simulink model "gtm_design_lpv"  (R2021b)
settings: Solver=VariableStepAuto  StartTime=0.0  StopTime=10  FixedStep=0.005  MaxStep=0.005  RelTol=1e-3
StopFcn:
  | MWSout=grabmws(bdroot);
  | MWSout.lastrun=datestr(now);
values from neighbouring files (symbols this model uses):
  s = tf('s')    [SingleDOF.m]    (also in main.m; mainSimple.m; newmain.m)
undefined symbols (not defined in the file or in its folder): Aero, aftfuel, aftfuel_pos, AILL, AILLC, AILR, AILRC, alpha_deg, altitude_ft, Ax_g, Ay_g, Az_g, b, beta_deg, bias, BRAKEC, Cbar, cg_pos0, cg_shift_gear, DamageCase, DamageModels, DamageOnsetTime, Earth, ELLIB, ELLIBC, ELLOB, ELLOBC, ELRIB, ELRIBC, ELROB, ELROBC, engl_ang, engl_pos, engr_ang, engr_pos, FLAPLIB, FLAPLIC, FLAPLOB, FLAPLOC, FLAPRIB, FLAPRIC, FLAPROB, FLAPROC, ft, FuelUsed_Init, fwdfuel, fwdfuel_pos, GEAR, GEARC, Inertia0, Inertia_shift_gear, Ixx_model, Iyy_model, Izz_model, KTAS, LandingGear, LengON, LinearizeModeOn, NAV_altitude_m, NAV_latitude_deg ... (+51)
libraries: simulink_extras x63, simulink_need_slupdate x30, LPVBlockLibrary x20, aerolibconvert2 x6, aerolibtransform2 x5, uavalgslib x4, UserContent_lib x3, simulink x3, robotcorelib x1, uavutilslib x1
(part 3 of 8)

== system gtm_design_lpv/Subsystem2/LPV1 ==
  Guidance : Inport
  Feedback : Inport  Port=2
  Add : Sum
  Bus Selector : BusSelector  OutputSignals=AirData.KTAS,AirData.altitude_ft,SurfacePos.AILL,SurfacePos.AILR
  Bus Selector3 : BusSelector  OutputSignals=An_c  OutputAsBus=on
  Bus Selector4 : BusSelector  OutputSignals=beta_c,phi_c  OutputAsBus=on
  Bus Selector5 : BusSelector  OutputSignals=AirData.alpha_deg,MAG3.q_deg,MAG3.Az_g
  Bus Selector6 : BusSelector  OutputSignals=AirData.beta_deg,MAG3.p_deg,MAG3.r_deg,MIDG.phi_deg,MAG3.Ay_g
  Bus to Vector : BusToVector
  Bus to Vector1 : BusToVector
  Constant : Constant
  Degrees to Radians{,1..5} (6 alike) : simulink_extras/Transformations/Degrees to Radians
  Demux1 : Demux  Outputs=2
  Gain : Gain  Gain=1/2
  Gain1 : Gain  Gain=1/100
  Gain2 : Gain  Gain=32.17405
  Gain3 : Gain  Gain=32.17405
  Gain4 : Gain  Gain=100
  Gain5 : Gain  Gain=100
  LPVBlock1 : LPVBlockLibrary/LPVBlock  sys=K_lon_lpv  plist={'rho1_tas_param';'rho2_alt_param';'rho3_mor_param'}  x0=0
      settings: SourceProductName=LPVTools Blocks
  LPVBlock2 : LPVBlockLibrary/LPVBlock  sys=K_lat_lpv  plist={'rho1_tas_param';'rho2_alt_param';'rho3_mor_param'}  x0=0
      settings: SourceProductName=LPVTools Blocks
  LPVBlock3 : LPVBlockLibrary/LPVBlock  sys=sch_alp_trim  plist={'rho1_tas_param';'rho2_alt_param';'rho3_mor_param'}  x0=0
      settings: SourceProductName=LPVTools Blocks
  Mux : Mux  Inputs=3
  Mux4 : Mux  Inputs=3
  Mux5 : Mux  Inputs=2
  Mux6 : Mux  Inputs=5
  Mux7 : Mux  Inputs=2
  Mux8 : Mux
  Radians to Degrees : simulink_extras/Transformations/Radians to Degrees
  Radians to Degrees1 : simulink_extras/Transformations/Radians to Degrees
  Selector : Selector  InputPortWidth=3  IndexOptions=Index vector (dialog)  Indices=3  OutputSizes=1
  Sum : Sum  Inputs=|+-
  Sum1 : Sum  Inputs=++|
  Sum2 : Sum  Inputs=|+-
  Out : Outport  InitialOutput=zeros(4,1)
  wires:
  Mux8/1 -> Out/1
  Radians to Degrees1/1 -> Mux8/1
  Gain4/1 -> Mux8/2
  Gain5/1 -> Mux8/3
  Radians to Degrees/1 -> Mux8/4
  Demux1/2 -> Radians to Degrees/1
  Sum1/1 -> Gain5/1
  Sum2/1 -> Gain4/1
  Demux1/1 -> Sum2/1, Sum1/2
  Selector/1 -> Sum2/2, Sum1/1
  [rho] -> Selector/1
  LPVBlock1/1 -> Radians to Degrees1/1
  LPVBlock2/1 -> Demux1/1
  [rho] -> LPVBlock2/2
  Mux7/1 -> LPVBlock2/1
  Bus to Vector1/1 -> Mux7/1
  Mux6/1 -> Mux7/2
  Degrees to Radians5/1 -> Mux6/4
  Degrees to Radians4/1 -> Mux6/3
  Degrees to Radians3/1 -> Mux6/2
  Degrees to Radians2/1 -> Mux6/1
  Gain3/1 -> Mux6/5
  Bus Selector6/5 -> Gain3/1  "<Ay_g>"
  Bus Selector6/4 -> Degrees to Radians5/1  "<phi_deg>"
  Bus Selector6/3 -> Degrees to Radians4/1  "<r_deg>"
  Bus Selector6/2 -> Degrees to Radians3/1  "<p_deg>"
  Bus Selector6/1 -> Degrees to Radians2/1  "<beta_deg>"
  Gain2/1 -> Mux4/3
  Degrees to Radians1/1 -> Mux4/2
  Degrees to Radians/1 -> Mux4/1
  Sum/1 -> Degrees to Radians/1
  LPVBlock3/1 -> Sum/2
  Bus Selector5/2 -> Degrees to Radians1/1  "<q_deg>"
  [rho] -> LPVBlock3/2
  Constant/1 -> LPVBlock3/1
  [rho] -> LPVBlock1/2
  Mux5/1 -> LPVBlock1/1
  Bus to Vector/1 -> Mux5/1
  Mux4/1 -> Mux5/2
  Bus Selector5/3 -> Gain2/1  "<Az_g>"
  Bus Selector5/1 -> Sum/1  "<alpha_deg>"
  Bus Selector4/1 -> Bus to Vector1/1
  Bus Selector3/1 -> Bus to Vector/1
  Guidance/1 -> Bus Selector3/1, Bus Selector4/1
  Gain1/1 -> Mux/3
  Add/1 -> Gain/1
  Feedback/1 -> Bus Selector5/1, Bus Selector6/1, Bus Selector/1
  Bus Selector/1 -> Mux/1  "<KTAS>"
  Bus Selector/3 -> Add/1  "<AILL>"
  Bus Selector/4 -> Add/2  "<AILR>"
  Bus Selector/2 -> Mux/2  "<altitude_ft>"
  Gain/1 -> Gain1/1
  Mux/1 -> [rho]

== system gtm_design_lpv/Subsystem2/Throttle Controller ==
  Constant : Constant  Value=36.739425746701627
  Constant1 : Constant  Value=0
  Out1 : Outport
  wires:
  Constant1/1 -> Out1/1

== system gtm_design_lpv/GTM_T2/A//C parameters/Inertia//Mass//CG Shift ==
  note: Inertia "vector" = [Ixx Iyy Izz Ixz Iyz Ixy]
  gear : Inport
  fuel_used : Inport  Port=2
  DamageCase : Inport  Port=3
  Add : Sum
  Add1 : Sum  Inputs=++++
  Add2 : Sum  Inputs=+++
  Add3 : Sum  Inputs=-+
  DamageEffects : Subsystem
  Divide1 : Product  Inputs=/*
  FuelBurnEffects : Subsystem
  Gain : Gain  Gain=1/32.17405
  Reshape : Reshape
  Reshape1 : Reshape
  Switch : Switch  Threshold=0.5
  Switch1 : Switch  Threshold=0.5
  cg/weight : Subsystem
  "fuel cg shift, cg_pos0" : MATLAB Function  TreatAsAtomicUnit=on
  ixxb3 : Constant  Value=Inertia0
  ixxb7 : Constant  Value=w0
  xCG1 : Constant  Value=zeros(1,3)
  xCG3 : Constant  Value=Inertia_shift_gear
  xCG4 : Constant  Value=cg_shift_gear
  xCG5 : Constant  Value=zeros(1,6)
  Inertia : Outport
  mass : Outport  Port=2
  CG : Outport  Port=3
  wires:
  "fuel cg shift, cg_pos0"/1(y) -> Divide1/2
  Divide1/1 -> Add2/2
  Reshape1/1 -> Inertia/1
  Reshape/1 -> CG/1
  cg/weight/2(dweight) -> Add/1
  gear/1 -> Switch1/2, Switch/2
  cg/weight/1(dCG) -> Add2/1
  Add3/1 -> Add/2
  xCG1/1 -> Switch1/3
  xCG4/1 -> Switch1/1
  Switch1/1 -> Add2/3
  ixxb7/1 -> Add3/2
  Gain/1 -> mass/1
  Add2/1 -> Reshape/1
  Add/1 -> Divide1/1, Gain/1  "gwest"
  DamageCase/1 -> cg/weight/1(DamageCase), DamageEffects/1(In)
  DamageEffects/1(dInertia) -> Add1/3
  ixxb3/1 -> Add1/4
  fuel_used/1 -> "fuel cg shift, cg_pos0"/1(fuel_used), Add3/1, FuelBurnEffects/1(In)
  xCG5/1 -> Switch/3
  xCG3/1 -> Switch/1
  Add1/1 -> Reshape1/1
  Switch/1 -> Add1/1
  FuelBurnEffects/1(dInertia) -> Add1/2

== system gtm_design_lpv/GTM_T2/A//C parameters/TriggerDamage ==
  Clock : Clock
  DamgeCase : Constant  Value=DamageCase
  Switch : Switch  Threshold=DamageOnsetTime
  Zero : Constant  Value=0
  damagecase : Outport
  wires:
  Clock/1 -> Switch/2
  Switch/1 -> damagecase/1
  Zero/1 -> Switch/3
  DamgeCase/1 -> Switch/1

== system gtm_design_lpv/GTM_T2/Actuators/Acutator Dynamics ==
  In : Inport
  Brake : Saturate  UpperLimit=100  LowerLimit=0
  Bus Selector2 : BusSelector  OutputSignals=ELLOBC,ELLIBC,ELROBC,ELRIBC,AILLC,AILRC,RUDUPC,RUDLOC,SPLLIBC,SPLLOBC,SPLRIBC,SPLROBC,FLAPLIC,FLAPLOC,FLAPRIC,FLAPROC,GEARC,BRAKEC,THROTLC,THROTRC,STEERC
  ElevatorLIBServo : Subsystem  mask(Rate and Position Limited Servo){freq=5, RL=300, POS_hi=20, POS_lo=-30, Bias=bias.elevator}
      mask prompts: freq "Bandwidth, Hz"; RL "Rate Limit:"; POS_hi "Position Limit High:"; POS_lo "Position Limit Low:"; Bias "Bias Value:"
      mask help:
      | First order transfer function: w/(s+w), with rate and position limits
      | and output bias level.
      mask Display:
      | text(.48,.55,sprintf('%3.1f Hz\nBW',freq),'horizontalAlignment','center');
      | 
      | text(0.18,0.45,sprintf('|d/dt|\n<%0.1f',RL),'horizontalAlignment','center');
      | 
      | text(0.88,0.85,num2str(POS_hi),'horizontalAlignment', 'center');
      | text(0.88,0.2,num2str(POS_lo),'horizontalAlignment', 'center');
      | text(0.73,0.5,'P\nL');
      | 
      | 
      | plot([0.83 0.87 0.93 0.97],[0.4 0.4 0.6 0.6]);
      | plot([0.81 0.99],[0.5 0.5]);
      | plot([0.9 0.9],[0.3 0.7]);
      | plot([0.81 0.99 0.99 0.81 0.81],[0.3 0.3 0.7 0.7 0.3]);
  ElevatorLOBServo : Subsystem  mask(Rate and Position Limited Servo){freq=5, RL=300, POS_hi=20, POS_lo=-30, Bias=bias.elevator}
      mask prompts: freq "Bandwidth, Hz"; RL "Rate Limit:"; POS_hi "Position Limit High:"; POS_lo "Position Limit Low:"; Bias "Bias Value:"
      mask help:
      | First order transfer function: w/(s+w), with rate and position limits
      | and output bias level.
      mask Display:
      | text(.48,.55,sprintf('%3.1f Hz\nBW',freq),'horizontalAlignment','center');
      | 
      | text(0.18,0.45,sprintf('|d/dt|\n<%0.1f',RL),'horizontalAlignment','center');
      | 
      | text(0.88,0.85,num2str(POS_hi),'horizontalAlignment', 'center');
      | text(0.88,0.2,num2str(POS_lo),'horizontalAlignment', 'center');
      | text(0.73,0.5,'P\nL');
      | 
      | 
      | plot([0.83 0.87 0.93 0.97],[0.4 0.4 0.6 0.6]);
      | plot([0.81 0.99],[0.5 0.5]);
      | plot([0.9 0.9],[0.3 0.7]);
      | plot([0.81 0.99 0.99 0.81 0.81],[0.3 0.3 0.7 0.7 0.3]);
  ElevatorRIBServo : Subsystem  mask(Rate and Position Limited Servo){freq=5, RL=300, POS_hi=20, POS_lo=-30, Bias=bias.elevator}
      mask prompts: freq "Bandwidth, Hz"; RL "Rate Limit:"; POS_hi "Position Limit High:"; POS_lo "Position Limit Low:"; Bias "Bias Value:"
      mask help:
      | First order transfer function: w/(s+w), with rate and position limits
      | and output bias level.
      mask Display:
      | text(.48,.55,sprintf('%3.1f Hz\nBW',freq),'horizontalAlignment','center');
      | 
      | text(0.18,0.45,sprintf('|d/dt|\n<%0.1f',RL),'horizontalAlignment','center');
      | 
      | text(0.88,0.85,num2str(POS_hi),'horizontalAlignment', 'center');
      | text(0.88,0.2,num2str(POS_lo),'horizontalAlignment', 'center');
      | text(0.73,0.5,'P\nL');
      | 
      | 
      | plot([0.83 0.87 0.93 0.97],[0.4 0.4 0.6 0.6]);
      | plot([0.81 0.99],[0.5 0.5]);
      | plot([0.9 0.9],[0.3 0.7]);
      | plot([0.81 0.99 0.99 0.81 0.81],[0.3 0.3 0.7 0.7 0.3]);
  ElevatorROBServo : Subsystem  mask(Rate and Position Limited Servo){freq=5, RL=300, POS_hi=20, POS_lo=-30, Bias=bias.elevator}
      mask prompts: freq "Bandwidth, Hz"; RL "Rate Limit:"; POS_hi "Position Limit High:"; POS_lo "Position Limit Low:"; Bias "Bias Value:"
      mask help:
      | First order transfer function: w/(s+w), with rate and position limits
      | and output bias level.
      mask Display:
      | text(.48,.55,sprintf('%3.1f Hz\nBW',freq),'horizontalAlignment','center');
      | 
      | text(0.18,0.45,sprintf('|d/dt|\n<%0.1f',RL),'horizontalAlignment','center');
      | 
      | text(0.88,0.85,num2str(POS_hi),'horizontalAlignment', 'center');
      | text(0.88,0.2,num2str(POS_lo),'horizontalAlignment', 'center');
      | text(0.73,0.5,'P\nL');
      | 
      | 
      | plot([0.83 0.87 0.93 0.97],[0.4 0.4 0.6 0.6]);
      | plot([0.81 0.99],[0.5 0.5]);
      | plot([0.9 0.9],[0.3 0.7]);
      | plot([0.81 0.99 0.99 0.81 0.81],[0.3 0.3 0.7 0.7 0.3]);
  FlapLIBServo : Subsystem  mask(Rate and Position Limited Servo){freq=5, RL=300, POS_hi=30, POS_lo=0, Bias=bias.flaps}
      mask prompts: freq "Bandwidth, Hz"; RL "Rate Limit:"; POS_hi "Position Limit High:"; POS_lo "Position Limit Low:"; Bias "Bias Value:"
      mask help:
      | First order transfer function: w/(s+w), with rate and position limits
      | and output bias level.
      mask Display:
      | text(.48,.55,sprintf('%3.1f Hz\nBW',freq),'horizontalAlignment','center');
      | 
      | text(0.18,0.45,sprintf('|d/dt|\n<%0.1f',RL),'horizontalAlignment','center');
      | 
      | text(0.88,0.85,num2str(POS_hi),'horizontalAlignment', 'center');
      | text(0.88,0.2,num2str(POS_lo),'horizontalAlignment', 'center');
      | text(0.73,0.5,'P\nL');
      | 
      | 
      | plot([0.83 0.87 0.93 0.97],[0.4 0.4 0.6 0.6]);
      | plot([0.81 0.99],[0.5 0.5]);
      | plot([0.9 0.9],[0.3 0.7]);
      | plot([0.81 0.99 0.99 0.81 0.81],[0.3 0.3 0.7 0.7 0.3]);
  FlapLOBServo : Subsystem  mask(Rate and Position Limited Servo){freq=5, RL=300, POS_hi=30, POS_lo=0, Bias=bias.flaps}
      mask prompts: freq "Bandwidth, Hz"; RL "Rate Limit:"; POS_hi "Position Limit High:"; POS_lo "Position Limit Low:"; Bias "Bias Value:"
      mask help:
      | First order transfer function: w/(s+w), with rate and position limits
      | and output bias level.
      mask Display:
      | text(.48,.55,sprintf('%3.1f Hz\nBW',freq),'horizontalAlignment','center');
      | 
      | text(0.18,0.45,sprintf('|d/dt|\n<%0.1f',RL),'horizontalAlignment','center');
      | 
      | text(0.88,0.85,num2str(POS_hi),'horizontalAlignment', 'center');
      | text(0.88,0.2,num2str(POS_lo),'horizontalAlignment', 'center');
      | text(0.73,0.5,'P\nL');
      | 
      | 
      | plot([0.83 0.87 0.93 0.97],[0.4 0.4 0.6 0.6]);
      | plot([0.81 0.99],[0.5 0.5]);
      | plot([0.9 0.9],[0.3 0.7]);
      | plot([0.81 0.99 0.99 0.81 0.81],[0.3 0.3 0.7 0.7 0.3]);
  FlapRIBServo : Subsystem  mask(Rate and Position Limited Servo){freq=5, RL=300, POS_hi=30, POS_lo=0, Bias=bias.flaps}
      mask prompts: freq "Bandwidth, Hz"; RL "Rate Limit:"; POS_hi "Position Limit High:"; POS_lo "Position Limit Low:"; Bias "Bias Value:"
      mask help:
      | First order transfer function: w/(s+w), with rate and position limits
      | and output bias level.
      mask Display:
      | text(.48,.55,sprintf('%3.1f Hz\nBW',freq),'horizontalAlignment','center');
      | 
      | text(0.18,0.45,sprintf('|d/dt|\n<%0.1f',RL),'horizontalAlignment','center');
      | 
      | text(0.88,0.85,num2str(POS_hi),'horizontalAlignment', 'center');
      | text(0.88,0.2,num2str(POS_lo),'horizontalAlignment', 'center');
      | text(0.73,0.5,'P\nL');
      | 
      | 
      | plot([0.83 0.87 0.93 0.97],[0.4 0.4 0.6 0.6]);
      | plot([0.81 0.99],[0.5 0.5]);
      | plot([0.9 0.9],[0.3 0.7]);
      | plot([0.81 0.99 0.99 0.81 0.81],[0.3 0.3 0.7 0.7 0.3]);
  FlapROBServo : Subsystem  mask(Rate and Position Limited Servo){freq=5, RL=300, POS_hi=30, POS_lo=0, Bias=bias.flaps}
      mask prompts: freq "Bandwidth, Hz"; RL "Rate Limit:"; POS_hi "Position Limit High:"; POS_lo "Position Limit Low:"; Bias "Bias Value:"
      mask help:
      | First order transfer function: w/(s+w), with rate and position limits
      | and output bias level.
      mask Display:
      | text(.48,.55,sprintf('%3.1f Hz\nBW',freq),'horizontalAlignment','center');
      | 
      | text(0.18,0.45,sprintf('|d/dt|\n<%0.1f',RL),'horizontalAlignment','center');
      | 
      | text(0.88,0.85,num2str(POS_hi),'horizontalAlignment', 'center');
      | text(0.88,0.2,num2str(POS_lo),'horizontalAlignment', 'center');
      | text(0.73,0.5,'P\nL');
      | 
      | 
      | plot([0.83 0.87 0.93 0.97],[0.4 0.4 0.6 0.6]);
      | plot([0.81 0.99],[0.5 0.5]);
      | plot([0.9 0.9],[0.3 0.7]);
      | plot([0.81 0.99 0.99 0.81 0.81],[0.3 0.3 0.7 0.7 0.3]);
  Gear : Saturate  UpperLimit=1  LowerLimit=0
  L Throttle : Saturate  UpperLimit=100  LowerLimit=0
  LeftAileronServo : Subsystem  mask(Rate and Position Limited Servo){freq=5, RL=300, POS_hi=0, POS_lo=-25, Bias=bias.morphing-bias.aileron}
      mask prompts: freq "Bandwidth, Hz"; RL "Rate Limit:"; POS_hi "Position Limit High:"; POS_lo "Position Limit Low:"; Bias "Bias Value:"
      mask help:
      | First order transfer function: w/(s+w), with rate and position limits
      | and output bias level.
      mask Display:
      | text(.48,.55,sprintf('%3.1f Hz\nBW',freq),'horizontalAlignment','center');
      | 
      | text(0.18,0.45,sprintf('|d/dt|\n<%0.1f',RL),'horizontalAlignment','center');
      | 
      | text(0.88,0.85,num2str(POS_hi),'horizontalAlignment', 'center');
      | text(0.88,0.2,num2str(POS_lo),'horizontalAlignment', 'center');
      | text(0.73,0.5,'P\nL');
      | 
      | 
      | plot([0.83 0.87 0.93 0.97],[0.4 0.4 0.6 0.6]);
      | plot([0.81 0.99],[0.5 0.5]);
      | plot([0.9 0.9],[0.3 0.7]);
      | plot([0.81 0.99 0.99 0.81 0.81],[0.3 0.3 0.7 0.7 0.3]);
  LeftIBSpoilerServo : Subsystem  mask(Rate and Position Limited Servo){freq=5, RL=300, POS_hi=15, POS_lo=0, Bias=bias.speedbrake}
      mask prompts: freq "Bandwidth, Hz"; RL "Rate Limit:"; POS_hi "Position Limit High:"; POS_lo "Position Limit Low:"; Bias "Bias Value:"
      mask help:
      | First order transfer function: w/(s+w), with rate and position limits
      | and output bias level.
      mask Display:
      | text(.48,.55,sprintf('%3.1f Hz\nBW',freq),'horizontalAlignment','center');
      | 
      | text(0.18,0.45,sprintf('|d/dt|\n<%0.1f',RL),'horizontalAlignment','center');
      | 
      | text(0.88,0.85,num2str(POS_hi),'horizontalAlignment', 'center');
      | text(0.88,0.2,num2str(POS_lo),'horizontalAlignment', 'center');
      | text(0.73,0.5,'P\nL');
      | 
      | 
      | plot([0.83 0.87 0.93 0.97],[0.4 0.4 0.6 0.6]);
      | plot([0.81 0.99],[0.5 0.5]);
      | plot([0.9 0.9],[0.3 0.7]);
      | plot([0.81 0.99 0.99 0.81 0.81],[0.3 0.3 0.7 0.7 0.3]);
  LeftOBSpoilerServo : Subsystem  mask(Rate and Position Limited Servo){freq=5, RL=300, POS_hi=45, POS_lo=0, Bias=bias.speedbrake}
      mask prompts: freq "Bandwidth, Hz"; RL "Rate Limit:"; POS_hi "Position Limit High:"; POS_lo "Position Limit Low:"; Bias "Bias Value:"
      mask help:
      | First order transfer function: w/(s+w), with rate and position limits
      | and output bias level.
      mask Display:
      | text(.48,.55,sprintf('%3.1f Hz\nBW',freq),'horizontalAlignment','center');
      | 
      | text(0.18,0.45,sprintf('|d/dt|\n<%0.1f',RL),'horizontalAlignment','center');
      | 
      | text(0.88,0.85,num2str(POS_hi),'horizontalAlignment', 'center');
      | text(0.88,0.2,num2str(POS_lo),'horizontalAlignment', 'center');
      | text(0.73,0.5,'P\nL');
      | 
      | 
      | plot([0.83 0.87 0.93 0.97],[0.4 0.4 0.6 0.6]);
      | plot([0.81 0.99],[0.5 0.5]);
      | plot([0.9 0.9],[0.3 0.7]);
      | plot([0.81 0.99 0.99 0.81 0.81],[0.3 0.3 0.7 0.7 0.3]);
  Mux : Mux  Inputs=21
  R Throttle : Saturate  UpperLimit=100  LowerLimit=0
  RightAileronServo : Subsystem  mask(Rate and Position Limited Servo){freq=5, RL=300, POS_hi=0, POS_lo=-25, Bias=bias.morphing+bias.aileron}
      mask prompts: freq "Bandwidth, Hz"; RL "Rate Limit:"; POS_hi "Position Limit High:"; POS_lo "Position Limit Low:"; Bias "Bias Value:"
      mask help:
      | First order transfer function: w/(s+w), with rate and position limits
      | and output bias level.
      mask Display:
      | text(.48,.55,sprintf('%3.1f Hz\nBW',freq),'horizontalAlignment','center');
      | 
      | text(0.18,0.45,sprintf('|d/dt|\n<%0.1f',RL),'horizontalAlignment','center');
      | 
      | text(0.88,0.85,num2str(POS_hi),'horizontalAlignment', 'center');
      | text(0.88,0.2,num2str(POS_lo),'horizontalAlignment', 'center');
      | text(0.73,0.5,'P\nL');
      | 
      | 
      | plot([0.83 0.87 0.93 0.97],[0.4 0.4 0.6 0.6]);
      | plot([0.81 0.99],[0.5 0.5]);
      | plot([0.9 0.9],[0.3 0.7]);
      | plot([0.81 0.99 0.99 0.81 0.81],[0.3 0.3 0.7 0.7 0.3]);
  RightIBSpoilerServo : Subsystem  mask(Rate and Position Limited Servo){freq=5, RL=300, POS_hi=15, POS_lo=0, Bias=bias.speedbrake}
      mask prompts: freq "Bandwidth, Hz"; RL "Rate Limit:"; POS_hi "Position Limit High:"; POS_lo "Position Limit Low:"; Bias "Bias Value:"
      mask help:
      | First order transfer function: w/(s+w), with rate and position limits
      | and output bias level.
      mask Display:
      | text(.48,.55,sprintf('%3.1f Hz\nBW',freq),'horizontalAlignment','center');
      | 
      | text(0.18,0.45,sprintf('|d/dt|\n<%0.1f',RL),'horizontalAlignment','center');
      | 
      | text(0.88,0.85,num2str(POS_hi),'horizontalAlignment', 'center');
      | text(0.88,0.2,num2str(POS_lo),'horizontalAlignment', 'center');
      | text(0.73,0.5,'P\nL');
      | 
      | 
      | plot([0.83 0.87 0.93 0.97],[0.4 0.4 0.6 0.6]);
      | plot([0.81 0.99],[0.5 0.5]);
      | plot([0.9 0.9],[0.3 0.7]);
      | plot([0.81 0.99 0.99 0.81 0.81],[0.3 0.3 0.7 0.7 0.3]);
  RightOBSpoilerServo : Subsystem  mask(Rate and Position Limited Servo){freq=5, RL=300, POS_hi=45, POS_lo=0, Bias=bias.speedbrake}
      mask prompts: freq "Bandwidth, Hz"; RL "Rate Limit:"; POS_hi "Position Limit High:"; POS_lo "Position Limit Low:"; Bias "Bias Value:"
      mask help:
      | First order transfer function: w/(s+w), with rate and position limits
      | and output bias level.
      mask Display:
      | text(.48,.55,sprintf('%3.1f Hz\nBW',freq),'horizontalAlignment','center');
      | 
      | text(0.18,0.45,sprintf('|d/dt|\n<%0.1f',RL),'horizontalAlignment','center');
      | 
      | text(0.88,0.85,num2str(POS_hi),'horizontalAlignment', 'center');
      | text(0.88,0.2,num2str(POS_lo),'horizontalAlignment', 'center');
      | text(0.73,0.5,'P\nL');
      | 
      | 
      | plot([0.83 0.87 0.93 0.97],[0.4 0.4 0.6 0.6]);
      | plot([0.81 0.99],[0.5 0.5]);
      | plot([0.9 0.9],[0.3 0.7]);
      | plot([0.81 0.99 0.99 0.81 0.81],[0.3 0.3 0.7 0.7 0.3]);
  RudderLServo : Subsystem  mask(Rate and Position Limited Servo){freq=5, RL=300, POS_hi=30, POS_lo=-30.0, Bias=bias.rudder}
      mask prompts: freq "Bandwidth, Hz"; RL "Rate Limit:"; POS_hi "Position Limit High:"; POS_lo "Position Limit Low:"; Bias "Bias Value:"
      mask help:
      | First order transfer function: w/(s+w), with rate and position limits
      | and output bias level.
      mask Display:
      | text(.48,.55,sprintf('%3.1f Hz\nBW',freq),'horizontalAlignment','center');
      | 
      | text(0.18,0.45,sprintf('|d/dt|\n<%0.1f',RL),'horizontalAlignment','center');
      | 
      | text(0.88,0.85,num2str(POS_hi),'horizontalAlignment', 'center');
      | text(0.88,0.2,num2str(POS_lo),'horizontalAlignment', 'center');
      | text(0.73,0.5,'P\nL');
      | 
      | 
      | plot([0.83 0.87 0.93 0.97],[0.4 0.4 0.6 0.6]);
      | plot([0.81 0.99],[0.5 0.5]);
      | plot([0.9 0.9],[0.3 0.7]);
      | plot([0.81 0.99 0.99 0.81 0.81],[0.3 0.3 0.7 0.7 0.3]);
  RudderUServo : Subsystem  mask(Rate and Position Limited Servo){freq=5, RL=300, POS_hi=30, POS_lo=-30.0, Bias=bias.rudder}
      mask prompts: freq "Bandwidth, Hz"; RL "Rate Limit:"; POS_hi "Position Limit High:"; POS_lo "Position Limit Low:"; Bias "Bias Value:"
      mask help:
      | First order transfer function: w/(s+w), with rate and position limits
      | and output bias level.
      mask Display:
      | text(.48,.55,sprintf('%3.1f Hz\nBW',freq),'horizontalAlignment','center');
      | 
      | text(0.18,0.45,sprintf('|d/dt|\n<%0.1f',RL),'horizontalAlignment','center');
      | 
      | text(0.88,0.85,num2str(POS_hi),'horizontalAlignment', 'center');
      | text(0.88,0.2,num2str(POS_lo),'horizontalAlignment', 'center');
      | text(0.73,0.5,'P\nL');
      | 
      | 
      | plot([0.83 0.87 0.93 0.97],[0.4 0.4 0.6 0.6]);
      | plot([0.81 0.99],[0.5 0.5]);
      | plot([0.9 0.9],[0.3 0.7]);
      | plot([0.81 0.99 0.99 0.81 0.81],[0.3 0.3 0.7 0.7 0.3]);
  Scope : Scope
  Scope1 : Scope
  Scope2 : Scope
  SteeringServo : Subsystem  mask(Rate and Position Limited Servo){freq=10, RL=300, POS_hi=30, POS_lo=-30, Bias=0}
      mask prompts: freq "Bandwidth, Hz"; RL "Rate Limit:"; POS_hi "Position Limit High:"; POS_lo "Position Limit Low:"; Bias "Bias Value:"
      mask help:
      | First order transfer function: w/(s+w), with rate and position limits
      | and output bias level.
      mask Display:
      | text(.48,.55,sprintf('%3.1f Hz\nBW',freq),'horizontalAlignment','center');
      | 
      | text(0.18,0.45,sprintf('|d/dt|\n<%0.1f',RL),'horizontalAlignment','center');
      | 
      | text(0.88,0.85,num2str(POS_hi),'horizontalAlignment', 'center');
      | text(0.88,0.2,num2str(POS_lo),'horizontalAlignment', 'center');
      | text(0.73,0.5,'P\nL');
      | 
      | 
      | plot([0.83 0.87 0.93 0.97],[0.4 0.4 0.6 0.6]);
      | plot([0.81 0.99],[0.5 0.5]);
      | plot([0.9 0.9],[0.3 0.7]);
      | plot([0.81 0.99 0.99 0.81 0.81],[0.3 0.3 0.7 0.7 0.3]);
  Sum : Sum  Inputs=++|
  Sum1 : Sum  Inputs=++|
  Sum2 : Sum  Inputs=++|
  Throttle : Constant  Value=bias.throttle
  Throttle1 : Constant  Value=bias.throttle
  Throttle2 : Constant  Value=bias.geardown
  Out : Outport
  wires:
  Bus Selector2/17 -> Sum2/2  "<GEARC>"
  Throttle2/1 -> Sum2/1
  Sum2/1 -> Gear/1
  Bus Selector2/20 -> Sum1/2  "<THROTRC>"
  Throttle1/1 -> Sum1/1
  Sum1/1 -> R Throttle/1
  Bus Selector2/19 -> Sum/2  "<THROTLC>"
  Throttle/1 -> Sum/1
  Sum/1 -> L Throttle/1
  SteeringServo/1(Out) -> Mux/21
  R Throttle/1 -> Mux/20
  L Throttle/1 -> Mux/19
  Brake/1 -> Mux/18
  Gear/1 -> Mux/17
  Mux/1 -> Out/1
  In/1 -> Bus Selector2/1
  Bus Selector2/21 -> SteeringServo/1(In)  "<STEERC>"
  FlapROBServo/1(Out) -> Mux/16
  FlapRIBServo/1(Out) -> Mux/15
  FlapLOBServo/1(Out) -> Mux/14
  FlapLIBServo/1(Out) -> Mux/13
  RightOBSpoilerServo/1(Out) -> Mux/12
  RightIBSpoilerServo/1(Out) -> Mux/11
  LeftOBSpoilerServo/1(Out) -> Mux/10
  LeftIBSpoilerServo/1(Out) -> Mux/9
  RudderLServo/1(Out) -> Mux/8
  Bus Selector2/12 -> RightOBSpoilerServo/1(In)  "<SPLROBC>"
  Bus Selector2/11 -> RightIBSpoilerServo/1(In)  "<SPLRIBC>"
  Bus Selector2/10 -> LeftOBSpoilerServo/1(In)  "<SPLLOBC>"
  Bus Selector2/9 -> LeftIBSpoilerServo/1(In)  "<SPLLIBC>"
  Bus Selector2/8 -> RudderLServo/1(In)  "<RUDLOC>"
  Bus Selector2/7 -> RudderUServo/1(In)  "<RUDUPC>"
  RudderUServo/1(Out) -> Scope2/1, Mux/7
  RightAileronServo/1(Out) -> Scope1/1, Mux/6
  Bus Selector2/6 -> RightAileronServo/1(In)  "<AILRC>"
  LeftAileronServo/1(Out) -> Mux/5
  Bus Selector2/5 -> LeftAileronServo/1(In)  "<AILLC>"
  ElevatorRIBServo/1(Out) -> Mux/4
  Bus Selector2/4 -> ElevatorRIBServo/1(In)  "<ELRIBC>"
  ElevatorROBServo/1(Out) -> Scope/1, Mux/3
  Bus Selector2/3 -> ElevatorROBServo/1(In)  "<ELROBC>"
  ElevatorLIBServo/1(Out) -> Mux/2
  ElevatorLOBServo/1(Out) -> Mux/1
  Bus Selector2/2 -> ElevatorLIBServo/1(In)  "<ELLIBC>"
  Bus Selector2/1 -> ElevatorLOBServo/1(In)  "<ELLOBC>"
  Bus Selector2/18 -> Brake/1  "<BRAKEC>"
  Bus Selector2/16 -> FlapROBServo/1(In)  "<FLAPROC>"
  Bus Selector2/15 -> FlapRIBServo/1(In)  "<FLAPRIC>"
  Bus Selector2/14 -> FlapLOBServo/1(In)  "<FLAPLOC>"
  Bus Selector2/13 -> FlapLIBServo/1(In)  "<FLAPLIC>"

== system gtm_design_lpv/GTM_T2/Actuators/Acutator Dynamics (Unbiased) ==
  note: Unbiased
  note: Unbiased
  In : Inport
  Brake : Saturate  UpperLimit=100  LowerLimit=0
  Bus Selector2 : BusSelector  OutputSignals=ELLOBC,ELLIBC,ELROBC,ELRIBC,AILLC,AILRC,RUDUPC,RUDLOC,SPLLIBC,SPLLOBC,SPLRIBC,SPLROBC,FLAPLIC,FLAPLOC,FLAPRIC,FLAPROC,GEARC,BRAKEC,THROTLC,THROTRC,STEERC
  ElevatorLIBServo : Subsystem  mask(Rate and Position Limited Servo){freq=5, RL=300, POS_hi=20, POS_lo=-30, Bias=0}
      mask prompts: freq "Bandwidth, Hz"; RL "Rate Limit:"; POS_hi "Position Limit High:"; POS_lo "Position Limit Low:"; Bias "Bias Value:"
      mask help:
      | First order transfer function: w/(s+w), with rate and position limits
      | and output bias level.
      mask Display:
      | text(.48,.55,sprintf('%3.1f Hz\nBW',freq),'horizontalAlignment','center');
      | 
      | text(0.18,0.45,sprintf('|d/dt|\n<%0.1f',RL),'horizontalAlignment','center');
      | 
      | text(0.88,0.85,num2str(POS_hi),'horizontalAlignment', 'center');
      | text(0.88,0.2,num2str(POS_lo),'horizontalAlignment', 'center');
      | text(0.73,0.5,'P\nL');
      | 
      | 
      | plot([0.83 0.87 0.93 0.97],[0.4 0.4 0.6 0.6]);
      | plot([0.81 0.99],[0.5 0.5]);
      | plot([0.9 0.9],[0.3 0.7]);
      | plot([0.81 0.99 0.99 0.81 0.81],[0.3 0.3 0.7 0.7 0.3]);
  ElevatorLOBServo : Subsystem  mask(Rate and Position Limited Servo){freq=5, RL=300, POS_hi=20, POS_lo=-30, Bias=0}
      mask prompts: freq "Bandwidth, Hz"; RL "Rate Limit:"; POS_hi "Position Limit High:"; POS_lo "Position Limit Low:"; Bias "Bias Value:"
      mask help:
      | First order transfer function: w/(s+w), with rate and position limits
      | and output bias level.
      mask Display:
      | text(.48,.55,sprintf('%3.1f Hz\nBW',freq),'horizontalAlignment','center');
      | 
      | text(0.18,0.45,sprintf('|d/dt|\n<%0.1f',RL),'horizontalAlignment','center');
      | 
      | text(0.88,0.85,num2str(POS_hi),'horizontalAlignment', 'center');
      | text(0.88,0.2,num2str(POS_lo),'horizontalAlignment', 'center');
      | text(0.73,0.5,'P\nL');
      | 
      | 
      | plot([0.83 0.87 0.93 0.97],[0.4 0.4 0.6 0.6]);
      | plot([0.81 0.99],[0.5 0.5]);
      | plot([0.9 0.9],[0.3 0.7]);
      | plot([0.81 0.99 0.99 0.81 0.81],[0.3 0.3 0.7 0.7 0.3]);
  ElevatorRIBServo : Subsystem  mask(Rate and Position Limited Servo){freq=5, RL=300, POS_hi=20, POS_lo=-30, Bias=0}
      mask prompts: freq "Bandwidth, Hz"; RL "Rate Limit:"; POS_hi "Position Limit High:"; POS_lo "Position Limit Low:"; Bias "Bias Value:"
      mask help:
      | First order transfer function: w/(s+w), with rate and position limits
      | and output bias level.
      mask Display:
      | text(.48,.55,sprintf('%3.1f Hz\nBW',freq),'horizontalAlignment','center');
      | 
      | text(0.18,0.45,sprintf('|d/dt|\n<%0.1f',RL),'horizontalAlignment','center');
      | 
      | text(0.88,0.85,num2str(POS_hi),'horizontalAlignment', 'center');
      | text(0.88,0.2,num2str(POS_lo),'horizontalAlignment', 'center');
      | text(0.73,0.5,'P\nL');
      | 
      | 
      | plot([0.83 0.87 0.93 0.97],[0.4 0.4 0.6 0.6]);
      | plot([0.81 0.99],[0.5 0.5]);
      | plot([0.9 0.9],[0.3 0.7]);
      | plot([0.81 0.99 0.99 0.81 0.81],[0.3 0.3 0.7 0.7 0.3]);
  ElevatorROBServo : Subsystem  mask(Rate and Position Limited Servo){freq=5, RL=300, POS_hi=20, POS_lo=-30, Bias=0}
      mask prompts: freq "Bandwidth, Hz"; RL "Rate Limit:"; POS_hi "Position Limit High:"; POS_lo "Position Limit Low:"; Bias "Bias Value:"
      mask help:
      | First order transfer function: w/(s+w), with rate and position limits
      | and output bias level.
      mask Display:
      | text(.48,.55,sprintf('%3.1f Hz\nBW',freq),'horizontalAlignment','center');
      | 
      | text(0.18,0.45,sprintf('|d/dt|\n<%0.1f',RL),'horizontalAlignment','center');
      | 
      | text(0.88,0.85,num2str(POS_hi),'horizontalAlignment', 'center');
      | text(0.88,0.2,num2str(POS_lo),'horizontalAlignment', 'center');
      | text(0.73,0.5,'P\nL');
      | 
      | 
      | plot([0.83 0.87 0.93 0.97],[0.4 0.4 0.6 0.6]);
      | plot([0.81 0.99],[0.5 0.5]);
      | plot([0.9 0.9],[0.3 0.7]);
      | plot([0.81 0.99 0.99 0.81 0.81],[0.3 0.3 0.7 0.7 0.3]);
  FlapLIBServo : Subsystem  mask(Rate and Position Limited Servo){freq=5, RL=300, POS_hi=30, POS_lo=0, Bias=bias.flaps}
      mask prompts: freq "Bandwidth, Hz"; RL "Rate Limit:"; POS_hi "Position Limit High:"; POS_lo "Position Limit Low:"; Bias "Bias Value:"
      mask help:
      | First order transfer function: w/(s+w), with rate and position limits
      | and output bias level.
      mask Display:
      | text(.48,.55,sprintf('%3.1f Hz\nBW',freq),'horizontalAlignment','center');
      | 
      | text(0.18,0.45,sprintf('|d/dt|\n<%0.1f',RL),'horizontalAlignment','center');
      | 
      | text(0.88,0.85,num2str(POS_hi),'horizontalAlignment', 'center');
      | text(0.88,0.2,num2str(POS_lo),'horizontalAlignment', 'center');
      | text(0.73,0.5,'P\nL');
      | 
      | 
      | plot([0.83 0.87 0.93 0.97],[0.4 0.4 0.6 0.6]);
      | plot([0.81 0.99],[0.5 0.5]);
      | plot([0.9 0.9],[0.3 0.7]);
      | plot([0.81 0.99 0.99 0.81 0.81],[0.3 0.3 0.7 0.7 0.3]);
  FlapLOBServo : Subsystem  mask(Rate and Position Limited Servo){freq=5, RL=300, POS_hi=30, POS_lo=0, Bias=bias.flaps}
      mask prompts: freq "Bandwidth, Hz"; RL "Rate Limit:"; POS_hi "Position Limit High:"; POS_lo "Position Limit Low:"; Bias "Bias Value:"
      mask help:
      | First order transfer function: w/(s+w), with rate and position limits
      | and output bias level.
      mask Display:
      | text(.48,.55,sprintf('%3.1f Hz\nBW',freq),'horizontalAlignment','center');
      | 
      | text(0.18,0.45,sprintf('|d/dt|\n<%0.1f',RL),'horizontalAlignment','center');
      | 
      | text(0.88,0.85,num2str(POS_hi),'horizontalAlignment', 'center');
      | text(0.88,0.2,num2str(POS_lo),'horizontalAlignment', 'center');
      | text(0.73,0.5,'P\nL');
      | 
      | 
      | plot([0.83 0.87 0.93 0.97],[0.4 0.4 0.6 0.6]);
      | plot([0.81 0.99],[0.5 0.5]);
      | plot([0.9 0.9],[0.3 0.7]);
      | plot([0.81 0.99 0.99 0.81 0.81],[0.3 0.3 0.7 0.7 0.3]);
  FlapRIBServo : Subsystem  mask(Rate and Position Limited Servo){freq=5, RL=300, POS_hi=30, POS_lo=0, Bias=bias.flaps}
      mask prompts: freq "Bandwidth, Hz"; RL "Rate Limit:"; POS_hi "Position Limit High:"; POS_lo "Position Limit Low:"; Bias "Bias Value:"
      mask help:
      | First order transfer function: w/(s+w), with rate and position limits
      | and output bias level.
      mask Display:
      | text(.48,.55,sprintf('%3.1f Hz\nBW',freq),'horizontalAlignment','center');
      | 
      | text(0.18,0.45,sprintf('|d/dt|\n<%0.1f',RL),'horizontalAlignment','center');
      | 
      | text(0.88,0.85,num2str(POS_hi),'horizontalAlignment', 'center');
      | text(0.88,0.2,num2str(POS_lo),'horizontalAlignment', 'center');
      | text(0.73,0.5,'P\nL');
      | 
      | 
      | plot([0.83 0.87 0.93 0.97],[0.4 0.4 0.6 0.6]);
      | plot([0.81 0.99],[0.5 0.5]);
      | plot([0.9 0.9],[0.3 0.7]);
      | plot([0.81 0.99 0.99 0.81 0.81],[0.3 0.3 0.7 0.7 0.3]);
  FlapROBServo : Subsystem  mask(Rate and Position Limited Servo){freq=5, RL=300, POS_hi=30, POS_lo=0, Bias=bias.flaps}
      mask prompts: freq "Bandwidth, Hz"; RL "Rate Limit:"; POS_hi "Position Limit High:"; POS_lo "Position Limit Low:"; Bias "Bias Value:"
      mask help:
      | First order transfer function: w/(s+w), with rate and position limits
      | and output bias level.
      mask Display:
      | text(.48,.55,sprintf('%3.1f Hz\nBW',freq),'horizontalAlignment','center');
      | 
      | text(0.18,0.45,sprintf('|d/dt|\n<%0.1f',RL),'horizontalAlignment','center');
      | 
      | text(0.88,0.85,num2str(POS_hi),'horizontalAlignment', 'center');
      | text(0.88,0.2,num2str(POS_lo),'horizontalAlignment', 'center');
      | text(0.73,0.5,'P\nL');
      | 
      | 
      | plot([0.83 0.87 0.93 0.97],[0.4 0.4 0.6 0.6]);
      | plot([0.81 0.99],[0.5 0.5]);
      | plot([0.9 0.9],[0.3 0.7]);
      | plot([0.81 0.99 0.99 0.81 0.81],[0.3 0.3 0.7 0.7 0.3]);
  Gear : Saturate  UpperLimit=1  LowerLimit=0
  L Throttle : Saturate  UpperLimit=100  LowerLimit=0
  LeftAileronServo : Subsystem  mask(Rate and Position Limited Servo){freq=5, RL=300, POS_hi=0, POS_lo=-25, Bias=0}
      mask prompts: freq "Bandwidth, Hz"; RL "Rate Limit:"; POS_hi "Position Limit High:"; POS_lo "Position Limit Low:"; Bias "Bias Value:"
      mask help:
      | First order transfer function: w/(s+w), with rate and position limits
      | and output bias level.
      mask Display:
      | text(.48,.55,sprintf('%3.1f Hz\nBW',freq),'horizontalAlignment','center');
      | 
      | text(0.18,0.45,sprintf('|d/dt|\n<%0.1f',RL),'horizontalAlignment','center');
      | 
      | text(0.88,0.85,num2str(POS_hi),'horizontalAlignment', 'center');
      | text(0.88,0.2,num2str(POS_lo),'horizontalAlignment', 'center');
      | text(0.73,0.5,'P\nL');
      | 
      | 
      | plot([0.83 0.87 0.93 0.97],[0.4 0.4 0.6 0.6]);
      | plot([0.81 0.99],[0.5 0.5]);
      | plot([0.9 0.9],[0.3 0.7]);
      | plot([0.81 0.99 0.99 0.81 0.81],[0.3 0.3 0.7 0.7 0.3]);
  LeftIBSpoilerServo : Subsystem  mask(Rate and Position Limited Servo){freq=5, RL=300, POS_hi=15, POS_lo=0, Bias=bias.speedbrake}
      mask prompts: freq "Bandwidth, Hz"; RL "Rate Limit:"; POS_hi "Position Limit High:"; POS_lo "Position Limit Low:"; Bias "Bias Value:"
      mask help:
      | First order transfer function: w/(s+w), with rate and position limits
      | and output bias level.
      mask Display:
      | text(.48,.55,sprintf('%3.1f Hz\nBW',freq),'horizontalAlignment','center');
      | 
      | text(0.18,0.45,sprintf('|d/dt|\n<%0.1f',RL),'horizontalAlignment','center');
      | 
      | text(0.88,0.85,num2str(POS_hi),'horizontalAlignment', 'center');
      | text(0.88,0.2,num2str(POS_lo),'horizontalAlignment', 'center');
      | text(0.73,0.5,'P\nL');
      | 
      | 
      | plot([0.83 0.87 0.93 0.97],[0.4 0.4 0.6 0.6]);
      | plot([0.81 0.99],[0.5 0.5]);
      | plot([0.9 0.9],[0.3 0.7]);
      | plot([0.81 0.99 0.99 0.81 0.81],[0.3 0.3 0.7 0.7 0.3]);
  LeftOBSpoilerServo : Subsystem  mask(Rate and Position Limited Servo){freq=5, RL=300, POS_hi=45, POS_lo=0, Bias=bias.speedbrake}
      mask prompts: freq "Bandwidth, Hz"; RL "Rate Limit:"; POS_hi "Position Limit High:"; POS_lo "Position Limit Low:"; Bias "Bias Value:"
      mask help:
      | First order transfer function: w/(s+w), with rate and position limits
      | and output bias level.
      mask Display:
      | text(.48,.55,sprintf('%3.1f Hz\nBW',freq),'horizontalAlignment','center');
      | 
      | text(0.18,0.45,sprintf('|d/dt|\n<%0.1f',RL),'horizontalAlignment','center');
      | 
      | text(0.88,0.85,num2str(POS_hi),'horizontalAlignment', 'center');
      | text(0.88,0.2,num2str(POS_lo),'horizontalAlignment', 'center');
      | text(0.73,0.5,'P\nL');
      | 
      | 
      | plot([0.83 0.87 0.93 0.97],[0.4 0.4 0.6 0.6]);
      | plot([0.81 0.99],[0.5 0.5]);
      | plot([0.9 0.9],[0.3 0.7]);
      | plot([0.81 0.99 0.99 0.81 0.81],[0.3 0.3 0.7 0.7 0.3]);
  Mux : Mux  Inputs=21
  R Throttle : Saturate  UpperLimit=100  LowerLimit=0
  RightAileronServo : Subsystem  mask(Rate and Position Limited Servo){freq=5, RL=300, POS_hi=0, POS_lo=-25, Bias=0}
      mask prompts: freq "Bandwidth, Hz"; RL "Rate Limit:"; POS_hi "Position Limit High:"; POS_lo "Position Limit Low:"; Bias "Bias Value:"
      mask help:
      | First order transfer function: w/(s+w), with rate and position limits
      | and output bias level.
      mask Display:
      | text(.48,.55,sprintf('%3.1f Hz\nBW',freq),'horizontalAlignment','center');
      | 
      | text(0.18,0.45,sprintf('|d/dt|\n<%0.1f',RL),'horizontalAlignment','center');
      | 
      | text(0.88,0.85,num2str(POS_hi),'horizontalAlignment', 'center');
      | text(0.88,0.2,num2str(POS_lo),'horizontalAlignment', 'center');
      | text(0.73,0.5,'P\nL');
      | 
      | 
      | plot([0.83 0.87 0.93 0.97],[0.4 0.4 0.6 0.6]);
      | plot([0.81 0.99],[0.5 0.5]);
      | plot([0.9 0.9],[0.3 0.7]);
      | plot([0.81 0.99 0.99 0.81 0.81],[0.3 0.3 0.7 0.7 0.3]);
  RightIBSpoilerServo : Subsystem  mask(Rate and Position Limited Servo){freq=5, RL=300, POS_hi=15, POS_lo=0, Bias=bias.speedbrake}
      mask prompts: freq "Bandwidth, Hz"; RL "Rate Limit:"; POS_hi "Position Limit High:"; POS_lo "Position Limit Low:"; Bias "Bias Value:"
      mask help:
      | First order transfer function: w/(s+w), with rate and position limits
      | and output bias level.
      mask Display:
      | text(.48,.55,sprintf('%3.1f Hz\nBW',freq),'horizontalAlignment','center');
      | 
      | text(0.18,0.45,sprintf('|d/dt|\n<%0.1f',RL),'horizontalAlignment','center');
      | 
      | text(0.88,0.85,num2str(POS_hi),'horizontalAlignment', 'center');
      | text(0.88,0.2,num2str(POS_lo),'horizontalAlignment', 'center');
      | text(0.73,0.5,'P\nL');
      | 
      | 
      | plot([0.83 0.87 0.93 0.97],[0.4 0.4 0.6 0.6]);
      | plot([0.81 0.99],[0.5 0.5]);
      | plot([0.9 0.9],[0.3 0.7]);
      | plot([0.81 0.99 0.99 0.81 0.81],[0.3 0.3 0.7 0.7 0.3]);
  RightOBSpoilerServo : Subsystem  mask(Rate and Position Limited Servo){freq=5, RL=300, POS_hi=45, POS_lo=0, Bias=bias.speedbrake}
      mask prompts: freq "Bandwidth, Hz"; RL "Rate Limit:"; POS_hi "Position Limit High:"; POS_lo "Position Limit Low:"; Bias "Bias Value:"
      mask help:
      | First order transfer function: w/(s+w), with rate and position limits
      | and output bias level.
      mask Display:
      | text(.48,.55,sprintf('%3.1f Hz\nBW',freq),'horizontalAlignment','center');
      | 
      | text(0.18,0.45,sprintf('|d/dt|\n<%0.1f',RL),'horizontalAlignment','center');
      | 
      | text(0.88,0.85,num2str(POS_hi),'horizontalAlignment', 'center');
      | text(0.88,0.2,num2str(POS_lo),'horizontalAlignment', 'center');
      | text(0.73,0.5,'P\nL');
      | 
      | 
      | plot([0.83 0.87 0.93 0.97],[0.4 0.4 0.6 0.6]);
      | plot([0.81 0.99],[0.5 0.5]);
      | plot([0.9 0.9],[0.3 0.7]);
      | plot([0.81 0.99 0.99 0.81 0.81],[0.3 0.3 0.7 0.7 0.3]);
  RudderLServo : Subsystem  mask(Rate and Position Limited Servo){freq=5, RL=300, POS_hi=30, POS_lo=-30.0, Bias=0}
      mask prompts: freq "Bandwidth, Hz"; RL "Rate Limit:"; POS_hi "Position Limit High:"; POS_lo "Position Limit Low:"; Bias "Bias Value:"
      mask help:
      | First order transfer function: w/(s+w), with rate and position limits
      | and output bias level.
      mask Display:
      | text(.48,.55,sprintf('%3.1f Hz\nBW',freq),'horizontalAlignment','center');
      | 
      | text(0.18,0.45,sprintf('|d/dt|\n<%0.1f',RL),'horizontalAlignment','center');
      | 
      | text(0.88,0.85,num2str(POS_hi),'horizontalAlignment', 'center');
      | text(0.88,0.2,num2str(POS_lo),'horizontalAlignment', 'center');
      | text(0.73,0.5,'P\nL');
      | 
      | 
      | plot([0.83 0.87 0.93 0.97],[0.4 0.4 0.6 0.6]);
      | plot([0.81 0.99],[0.5 0.5]);
      | plot([0.9 0.9],[0.3 0.7]);
      | plot([0.81 0.99 0.99 0.81 0.81],[0.3 0.3 0.7 0.7 0.3]);
  RudderUServo : Subsystem  mask(Rate and Position Limited Servo){freq=5, RL=300, POS_hi=30, POS_lo=-30.0, Bias=0}
      mask prompts: freq "Bandwidth, Hz"; RL "Rate Limit:"; POS_hi "Position Limit High:"; POS_lo "Position Limit Low:"; Bias "Bias Value:"
      mask help:
      | First order transfer function: w/(s+w), with rate and position limits
      | and output bias level.
      mask Display:
      | text(.48,.55,sprintf('%3.1f Hz\nBW',freq),'horizontalAlignment','center');
      | 
      | text(0.18,0.45,sprintf('|d/dt|\n<%0.1f',RL),'horizontalAlignment','center');
      | 
      | text(0.88,0.85,num2str(POS_hi),'horizontalAlignment', 'center');
      | text(0.88,0.2,num2str(POS_lo),'horizontalAlignment', 'center');
      | text(0.73,0.5,'P\nL');
      | 
      | 
      | plot([0.83 0.87 0.93 0.97],[0.4 0.4 0.6 0.6]);
      | plot([0.81 0.99],[0.5 0.5]);
      | plot([0.9 0.9],[0.3 0.7]);
      | plot([0.81 0.99 0.99 0.81 0.81],[0.3 0.3 0.7 0.7 0.3]);
  SteeringServo : Subsystem  mask(Rate and Position Limited Servo){freq=10, RL=300, POS_hi=30, POS_lo=-30, Bias=0}
      mask prompts: freq "Bandwidth, Hz"; RL "Rate Limit:"; POS_hi "Position Limit High:"; POS_lo "Position Limit Low:"; Bias "Bias Value:"
      mask help:
      | First order transfer function: w/(s+w), with rate and position limits
      | and output bias level.
      mask Display:
      | text(.48,.55,sprintf('%3.1f Hz\nBW',freq),'horizontalAlignment','center');
      | 
      | text(0.18,0.45,sprintf('|d/dt|\n<%0.1f',RL),'horizontalAlignment','center');
      | 
      | text(0.88,0.85,num2str(POS_hi),'horizontalAlignment', 'center');
      | text(0.88,0.2,num2str(POS_lo),'horizontalAlignment', 'center');
      | text(0.73,0.5,'P\nL');
      | 
      | 
      | plot([0.83 0.87 0.93 0.97],[0.4 0.4 0.6 0.6]);
      | plot([0.81 0.99],[0.5 0.5]);
      | plot([0.9 0.9],[0.3 0.7]);
      | plot([0.81 0.99 0.99 0.81 0.81],[0.3 0.3 0.7 0.7 0.3]);
  Sum : Sum  Inputs=++|
  Sum1 : Sum  Inputs=++|
  Sum2 : Sum  Inputs=++|
  Throttle : Constant  Value=0
  Throttle1 : Constant  Value=0
  Throttle2 : Constant  Value=bias.geardown
  Out : Outport
  wires:
  Bus Selector2/13 -> FlapLIBServo/1(In)  "<FLAPLIC>"
  Bus Selector2/14 -> FlapLOBServo/1(In)  "<FLAPLOC>"
  Bus Selector2/15 -> FlapRIBServo/1(In)  "<FLAPRIC>"
  Bus Selector2/16 -> FlapROBServo/1(In)  "<FLAPROC>"
  Bus Selector2/18 -> Brake/1  "<BRAKEC>"
  Bus Selector2/1 -> ElevatorLOBServo/1(In)  "<ELLOBC>"
  Bus Selector2/2 -> ElevatorLIBServo/1(In)  "<ELLIBC>"
  ElevatorLOBServo/1(Out) -> Mux/1
  ElevatorLIBServo/1(Out) -> Mux/2
  Bus Selector2/3 -> ElevatorROBServo/1(In)  "<ELROBC>"
  ElevatorROBServo/1(Out) -> Mux/3
  Bus Selector2/4 -> ElevatorRIBServo/1(In)  "<ELRIBC>"
  ElevatorRIBServo/1(Out) -> Mux/4
  Bus Selector2/5 -> LeftAileronServo/1(In)  "<AILLC>"
  LeftAileronServo/1(Out) -> Mux/5
  Bus Selector2/6 -> RightAileronServo/1(In)  "<AILRC>"
  RightAileronServo/1(Out) -> Mux/6
  RudderUServo/1(Out) -> Mux/7
  Bus Selector2/7 -> RudderUServo/1(In)  "<RUDUPC>"
  Bus Selector2/8 -> RudderLServo/1(In)  "<RUDLOC>"
  Bus Selector2/9 -> LeftIBSpoilerServo/1(In)  "<SPLLIBC>"
  Bus Selector2/10 -> LeftOBSpoilerServo/1(In)  "<SPLLOBC>"
  Bus Selector2/11 -> RightIBSpoilerServo/1(In)  "<SPLRIBC>"
  Bus Selector2/12 -> RightOBSpoilerServo/1(In)  "<SPLROBC>"
  RudderLServo/1(Out) -> Mux/8
  LeftIBSpoilerServo/1(Out) -> Mux/9
  LeftOBSpoilerServo/1(Out) -> Mux/10
  RightIBSpoilerServo/1(Out) -> Mux/11
  RightOBSpoilerServo/1(Out) -> Mux/12
  FlapLIBServo/1(Out) -> Mux/13
  FlapLOBServo/1(Out) -> Mux/14
  FlapRIBServo/1(Out) -> Mux/15
  FlapROBServo/1(Out) -> Mux/16
  Bus Selector2/21 -> SteeringServo/1(In)  "<STEERC>"
  In/1 -> Bus Selector2/1
  Mux/1 -> Out/1
  Gear/1 -> Mux/17
  Brake/1 -> Mux/18
  L Throttle/1 -> Mux/19
  R Throttle/1 -> Mux/20
  SteeringServo/1(Out) -> Mux/21
  Sum/1 -> L Throttle/1
  Throttle/1 -> Sum/1
  Bus Selector2/19 -> Sum/2  "<THROTLC>"
  Sum1/1 -> R Throttle/1
  Throttle1/1 -> Sum1/1
  Bus Selector2/20 -> Sum1/2  "<THROTRC>"
  Sum2/1 -> Gear/1
  Throttle2/1 -> Sum2/1
  Bus Selector2/17 -> Sum2/2  "<GEARC>"

== system gtm_design_lpv/GTM_T2/Actuators/DeadBand ==
  I : Inport
  Deadband : Subsystem
  Flaps : Constant  Value=SurfaceDeadbandOn
  Switch : Switch  Criteria=u2 ~= 0  Threshold=0.2
  O : Outport
  wires:
  I/1 -> Switch/3, Deadband/1(In)
  Deadband/1(Out) -> Switch/1
  Switch/1 -> O/1
  Flaps/1 -> Switch/2

== system gtm_design_lpv/GTM_T2/Actuators/InputModification for Trimming ==
  CmdVec : Inport
  SurfBias : Inport  Port=2
  SurfaceDeltas : Inport  Port=3
  Clock : Clock
  Compare To Constant : simulink/Logic and Bit Operations/Compare To Constant  relop=>=  const=0.2  OutDataTypeStr=boolean  ZeroCross=off
  Constant : Constant  Value=TrimModeOn
  Constant1 : Constant  Value=LinearizeModeOn
  Constant2 : Constant  Value=TrimModeOn
  Constant3 : Constant  Value=LinearizeModeOn
  Gain : Gain  Gain=2
  "Invalid, Error Out" : Subsystem  TreatAsAtomicUnit=on
  KillifNotSimMode : Assertion  AssertionFailFcn="warndlg('Running simulation with TrimMode or LinearizeMode engaged.  Run setup.m to reset.','Warning!')"
  LinearizeMode:DetlasOnTrimBias : Subsystem  TreatAsAtomicUnit=on
  Logical Operator : Logic  Operator=NAND  AllPortsSameDT=off  OutDataTypeStr=boolean
  Logical Operator1 : Logic  Operator=OR  AllPortsSameDT=off  OutDataTypeStr=boolean
  Merge : Merge  Inputs=4  InitialOutput=zeros(22,1)
  SimMode:PassThroughWithStab : Subsystem  TreatAsAtomicUnit=on
  Sum : Sum  Inputs=|++
  Switch Case : SwitchCase  CaseConditions={0,1,2}
  TrimMode: DriveFromTopLevel : Subsystem  TreatAsAtomicUnit=on
  CmdVecOut : Outport
  wires:
  "Invalid, Error Out"/1(Out) -> Merge/4
  Compare To Constant/1 -> Logical Operator/2
  Logical Operator1/1 -> Logical Operator/1
  Constant2/1 -> Logical Operator1/1
  Constant3/1 -> Logical Operator1/2
  Logical Operator/1 -> KillifNotSimMode/1
  Clock/1 -> Compare To Constant/1
  Switch Case/4 -> "Invalid, Error Out"/Action
  Sum/1 -> Switch Case/1
  Gain/1 -> Sum/2
  Constant/1 -> Sum/1
  Constant1/1 -> Gain/1
  LinearizeMode:DetlasOnTrimBias/1(Out) -> Merge/3
  SurfaceDeltas/1 -> LinearizeMode:DetlasOnTrimBias/1(In1)
  Switch Case/3 -> LinearizeMode:DetlasOnTrimBias/Action
  Merge/1 -> CmdVecOut/1
  TrimMode: DriveFromTopLevel/1(Out) -> Merge/2
  SimMode:PassThroughWithStab/1(Out) -> Merge/1
  SurfBias/1 -> TrimMode: DriveFromTopLevel/1(TrimBias)
  Switch Case/2 -> TrimMode: DriveFromTopLevel/Action
  Switch Case/1 -> SimMode:PassThroughWithStab/Action
  CmdVec/1 -> SimMode:PassThroughWithStab/1(Cmd)

== system gtm_design_lpv/GTM_T2/Actuators/Label ==
  I : Inport
  Bus Creator : BusCreator  Inputs=22
  Demux : Demux  Outputs=22
  O : Outport
  wires:
  Demux/22 -> Bus Creator/22  "STEER"
  Demux/21 -> Bus Creator/21  "THROTR"
  Demux/20 -> Bus Creator/20  "THROTL"
  Demux/19 -> Bus Creator/19  "BRAKE"
  Demux/1 -> Bus Creator/1  "ELLOB"
  Demux/18 -> Bus Creator/18  "GEAR"
  Demux/17 -> Bus Creator/17  "STAB"
  Demux/16 -> Bus Creator/16  "FLAPROB"
  Demux/15 -> Bus Creator/15  "FLAPRIB"
  Demux/14 -> Bus Creator/14  "FLAPLOB"
  Demux/13 -> Bus Creator/13  "FLAPLIB"
  Demux/12 -> Bus Creator/12  "SPLROB"
  Demux/11 -> Bus Creator/11  "SPLRIB"
  Demux/10 -> Bus Creator/10  "SPLLOB"
  Demux/9 -> Bus Creator/9  "SPLLIB"
  Demux/8 -> Bus Creator/8  "RUDL"
  Demux/7 -> Bus Creator/7  "RUDU"
  Demux/6 -> Bus Creator/6  "AILR"
  Demux/5 -> Bus Creator/5  "AILL"
  Demux/4 -> Bus Creator/4  "ELRIB"
  Demux/3 -> Bus Creator/3  "ELROB"
  Demux/2 -> Bus Creator/2  "ELLIB"
  Bus Creator/1 -> O/1
  I/1 -> Demux/1

== system gtm_design_lpv/GTM_T2/Actuators/TimeDelay with IC feedthrough ==
  I : Inport
  Clock : Clock
  Demux : Demux  Outputs=[16 5]
  Mux : Mux  Inputs=[16 5]
  Switch : Switch  Threshold=10.1e-3
  Transport Delay : TransportDelay  DelayTime=10e-3
      settings: AttributesFormatString=%<DelayTime>
  O : Outport
  wires:
  Mux/1 -> Switch/1
  Demux/2 -> Mux/2
  Transport Delay/1 -> Mux/1
  Demux/1 -> Transport Delay/1
  Switch/1 -> O/1
  Clock/1 -> Switch/2
  I/1 -> Demux/1, Switch/3
